simulink model "BLDC_ClosedLoop"  (R2025a)
settings: Solver=FixedStepDiscrete  StartTime=0.0  StopTime=Tsim  FixedStep=Ts  RelTol=1e-3
undefined symbols (not defined in the file): antiWindupEnable, B, DiscIntNeverNeededParam, fPWM, J, Ki, Kp, Ls, polePairs, refSpeed1, refSpeed2, refTime1, refTime2, Rs, speedRampRate, TloadInitial, TloadStep, TloadStepTime, Ts, Ts_speed, uMax, uMin, Vdc
libraries: simulink x7, spsPermanentMagnetSynchronousMachineLib x1, spsControlledVoltageSourceLib x1, spsUniversalBridgeLib x1, spsVoltageMeasurementLib x1, spspowerguiLib x1
settings Model: Creator=yegan  LastModifiedBy=yegan
settings SolverCC: AutoInsertRateTranBlk=on
settings DataIOCC: SaveOutput=off  SaveTime=off

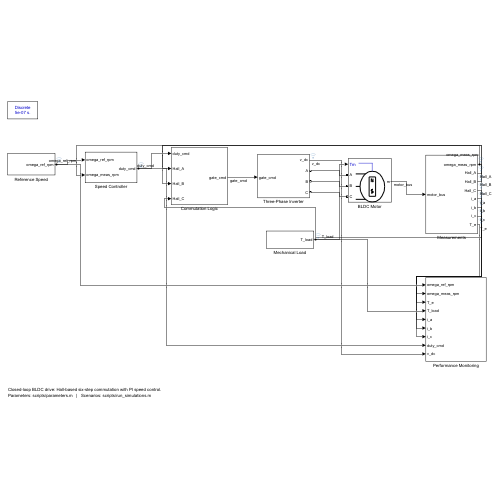
[thumbnail: Simulink's stored preview of the top-level diagram]
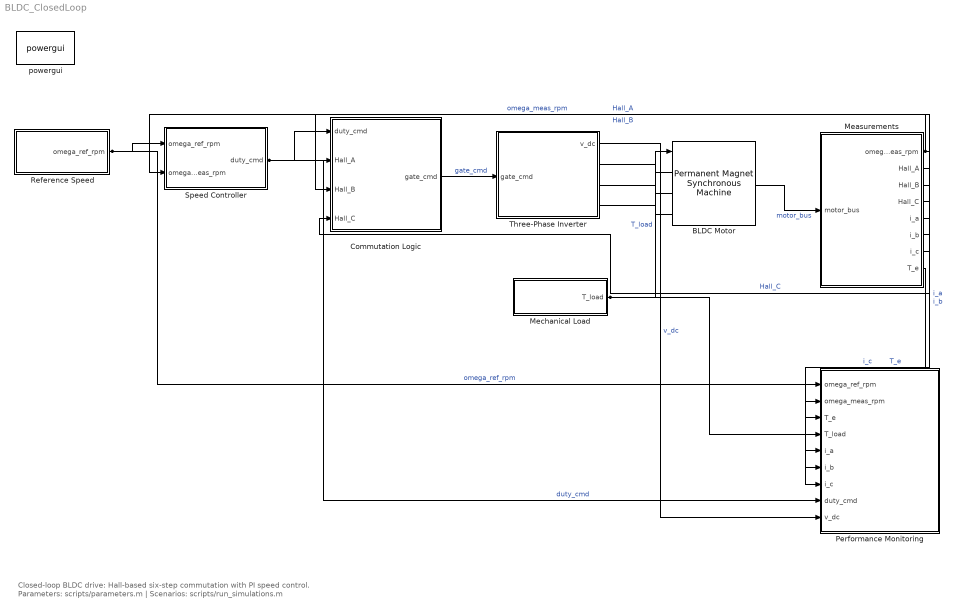
== system BLDC_ClosedLoop ==
  note: Closed-loop BLDC drive: Hall-based six-step commutation with PI speed control.
      | Parameters: scripts/parameters.m   |   Scenarios: scripts/run_simulations.m
  BLDC Motor : spsPermanentMagnetSynchronousMachineLib/Permanent Magnet Synchronous Machine  NbPhases=3  FluxDistribution=Trapezoidal  RotorType=Round  MechanicalLoad=Torque Tm  PresetModel=No  ShowDetailedParameters=on  MeasurementBus=off  Resistance=Rs  Inductance=Ls  dqInductances=[8.5e-3,8.5e-3]  La=0.000395  MachineConstant=Flux linkage established by magnets (V.s)  Flux=fluxPM  VoltageCst=87.9646  TorqueCst=0.84  Flat=flatTopDeg  Mechanical=[J, B, polePairs, 0]  PolePairs=polePairs  InitialConditions=[0, 0, 0, 0]  InitialConditions5ph=[0 0 0 0 0 0]  RefAngle=90 degrees behind phase A axis (modified Park)  IterativeDiscreteModel=Trapezoidal non iterative  TsBlock=-1  TsPowergui=0
  Commutation Logic : Subsystem
  Measurements : Subsystem
  Mechanical Load : Subsystem
  Performance Monitoring : Subsystem
  Reference Speed : Subsystem
  Speed Controller : Subsystem
  Three-Phase Inverter : Subsystem
  powergui : spspowerguiLib/powergui  Priority=1  SimulationMode=Discrete  SampleTime=Ts  frequency=60  Iterations=50  frequencyindice=60  Pbase=100e6  ErrMax=1e-4  UnitsV=kV  UnitsW=MW  buscounter=0  FunctionMessages=off  echomessages=off  EnableUseOfTLC=off  CurrentSourceSwitches=off  DisableSnubberDevices=off  DisableRonSwitches=off  DisableVfSwitches=off  DisplayEquations=off  AutomaticDiscreteSolvers=off  SolverType=Tustin/Backward Euler (TBE)  Interpol=off  ExternalGateDelay=off  methode=off  Ts=100  x0status=blocks  SPID=on  SwTol=0  HookPort=off  NonlinearTolerance=1e-4  nMaxIteration=100  ContinueOnMaxIteration=off  RestoreLinks=warning  ResistiveCurrentMeasurement=off  Frange=[0:2:500]  Ylog=off  Xlog=on  ShowGrid=off  save=off  variable=ZData  structure=0  ZoomFFT=off  StartTime=0.0  cycles=1  DisplayStyle=1  fundamental=60  FreqAxis=off  MaxFrequency=1000  frequencyindicesteady=1  RmsSteady=1  display=off
  wires:
  Reference Speed/1(omega_ref_rpm) -> Speed Controller/1(omega_ref_rpm), Performance Monitoring/1(omega_ref_rpm)  "omega_ref_rpm"
  Speed Controller/1(duty_cmd) -> Commutation Logic/1(duty_cmd), Performance Monitoring/8(duty_cmd)  "duty_cmd"
  Commutation Logic/1(gate_cmd) -> Three-Phase Inverter/1(gate_cmd)  "gate_cmd"
  Three-Phase Inverter/1(v_dc) -> Performance Monitoring/9(v_dc)  "v_dc"
  Mechanical Load/1(T_load) -> BLDC Motor/1, Performance Monitoring/4(T_load)  "T_load"
  BLDC Motor/1 -> Measurements/1(motor_bus)  "motor_bus"
  Measurements/1(omega_meas_rpm) -> Speed Controller/2(omega_meas_rpm), Performance Monitoring/2(omega_meas_rpm)  "omega_meas_rpm"
  Measurements/2(Hall_A) -> Commutation Logic/2(Hall_A)  "Hall_A"
  Measurements/3(Hall_B) -> Commutation Logic/3(Hall_B)  "Hall_B"
  Measurements/4(Hall_C) -> Commutation Logic/4(Hall_C)  "Hall_C"
  Measurements/5(i_a) -> Performance Monitoring/5(i_a)  "i_a"
  Measurements/6(i_b) -> Performance Monitoring/6(i_b)  "i_b"
  Measurements/7(i_c) -> Performance Monitoring/7(i_c)  "i_c"
  Measurements/8(T_e) -> Performance Monitoring/3(T_e)  "T_e"
  connections:
  Three-Phase Inverter/RConn1 -- BLDC Motor/LConn1
  Three-Phase Inverter/RConn2 -- BLDC Motor/LConn2
  Three-Phase Inverter/RConn3 -- BLDC Motor/LConn3

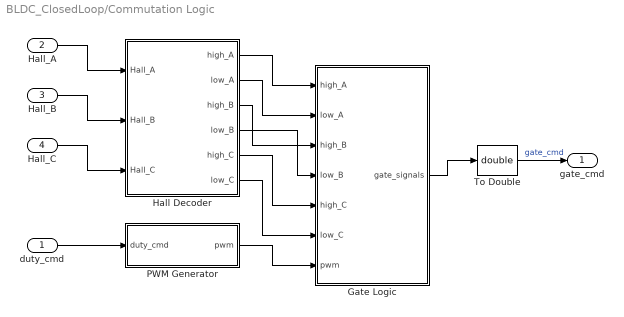
== system BLDC_ClosedLoop/Commutation Logic ==
  duty_cmd : Inport
  Hall_A : Inport  Port=2
  Hall_B : Inport  Port=3
  Hall_C : Inport  Port=4
  Gate Logic : Subsystem
  Hall Decoder : Subsystem
  PWM Generator : Subsystem
  To Double : DataTypeConversion  OutDataTypeStr=double  SaturateOnIntegerOverflow=off  RndMeth=Floor
  gate_cmd : Outport
  wires:
  Hall_A/1 -> Hall Decoder/1(Hall_A)
  Hall_B/1 -> Hall Decoder/2(Hall_B)
  Hall_C/1 -> Hall Decoder/3(Hall_C)
  duty_cmd/1 -> PWM Generator/1(duty_cmd)
  Hall Decoder/1(high_A) -> Gate Logic/1(high_A)
  Hall Decoder/2(low_A) -> Gate Logic/2(low_A)
  Hall Decoder/3(high_B) -> Gate Logic/3(high_B)
  Hall Decoder/4(low_B) -> Gate Logic/4(low_B)
  Hall Decoder/5(high_C) -> Gate Logic/5(high_C)
  Hall Decoder/6(low_C) -> Gate Logic/6(low_C)
  PWM Generator/1(pwm) -> Gate Logic/7(pwm)
  Gate Logic/1(gate_signals) -> To Double/1
  To Double/1 -> gate_cmd/1  "gate_cmd"

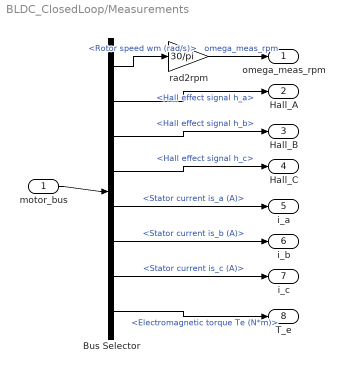
== system BLDC_ClosedLoop/Measurements ==
  motor_bus : Inport
  Bus Selector : BusSelector  OutputSignals=Rotor speed wm (rad/s),Hall effect signal h_a,Hall effect signal h_b,Hall effect signal h_c,Stator current is_a (A),Stator current is_b (A),Stator current is_c (A),Electromagnetic torque Te (N*m)
  rad2rpm : Gain  Gain=30/pi
  omega_meas_rpm : Outport
  Hall_A : Outport  Port=2
  Hall_B : Outport  Port=3
  Hall_C : Outport  Port=4
  i_a : Outport  Port=5
  i_b : Outport  Port=6
  i_c : Outport  Port=7
  T_e : Outport  Port=8
  wires:
  motor_bus/1 -> Bus Selector/1
  Bus Selector/1 -> rad2rpm/1  "<Rotor speed wm (rad/s)>"
  rad2rpm/1 -> omega_meas_rpm/1  "omega_meas_rpm"
  Bus Selector/2 -> Hall_A/1  "<Hall effect signal h_a>"
  Bus Selector/3 -> Hall_B/1  "<Hall effect signal h_b>"
  Bus Selector/4 -> Hall_C/1  "<Hall effect signal h_c>"
  Bus Selector/5 -> i_a/1  "<Stator current is_a (A)>"
  Bus Selector/6 -> i_b/1  "<Stator current is_b (A)>"
  Bus Selector/7 -> i_c/1  "<Stator current is_c (A)>"
  Bus Selector/8 -> T_e/1  "<Electromagnetic torque Te (N*m)>"

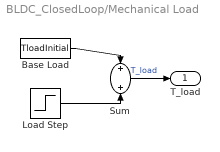
== system BLDC_ClosedLoop/Mechanical Load ==
  Base Load : Constant  Value=TloadInitial
  Load Step : Step  Time=TloadStepTime  After=TloadStep  SampleTime=0
  Sum : Sum
  T_load : Outport
  wires:
  Base Load/1 -> Sum/1
  Load Step/1 -> Sum/2
  Sum/1 -> T_load/1  "T_load"

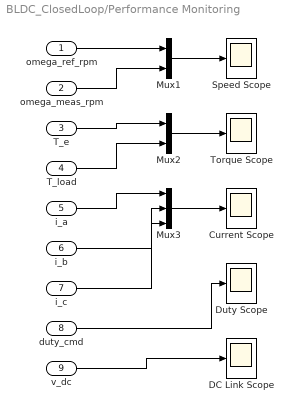
== system BLDC_ClosedLoop/Performance Monitoring ==
  omega_ref_rpm : Inport
  omega_meas_rpm : Inport  Port=2
  T_e : Inport  Port=3
  T_load : Inport  Port=4
  i_a : Inport  Port=5
  i_b : Inport  Port=6
  i_c : Inport  Port=7
  duty_cmd : Inport  Port=8
  v_dc : Inport  Port=9
  Current Scope : Scope
  DC Link Scope : Scope
  Duty Scope : Scope
  Mux1 : Mux  Inputs=2
  Mux2 : Mux  Inputs=2
  Mux3 : Mux  Inputs=3
  Speed Scope : Scope
  Torque Scope : Scope
  wires:
  omega_ref_rpm/1 -> Mux1/1
  omega_meas_rpm/1 -> Mux1/2
  Mux1/1 -> Speed Scope/1
  T_e/1 -> Mux2/1
  T_load/1 -> Mux2/2
  Mux2/1 -> Torque Scope/1
  i_a/1 -> Mux3/1
  i_b/1 -> Mux3/2
  i_c/1 -> Mux3/3
  Mux3/1 -> Current Scope/1
  duty_cmd/1 -> Duty Scope/1
  v_dc/1 -> DC Link Scope/1

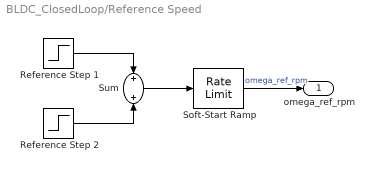
== system BLDC_ClosedLoop/Reference Speed ==
  Reference Step 1 : Step  Time=refTime1  After=refSpeed1  SampleTime=Ts_speed
  Reference Step 2 : Step  Time=refTime2  After=refSpeed2 - refSpeed1  SampleTime=Ts_speed
  Soft-Start Ramp : RateLimiter  RisingSlewLimit=speedRampRate  FallingSlewLimit=-speedRampRate  SampleTimeMode=inherited
  Sum : Sum
  omega_ref_rpm : Outport
  wires:
  Reference Step 1/1 -> Sum/1
  Reference Step 2/1 -> Sum/2
  Sum/1 -> Soft-Start Ramp/1
  Soft-Start Ramp/1 -> omega_ref_rpm/1  "omega_ref_rpm"

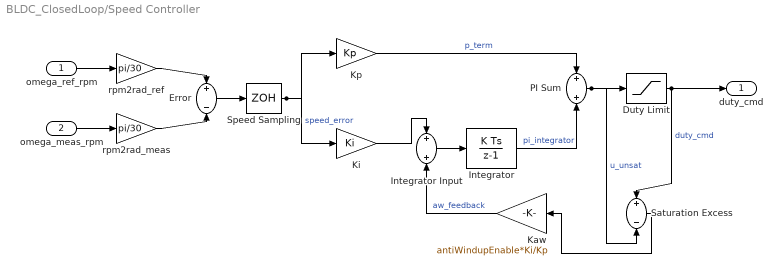
== system BLDC_ClosedLoop/Speed Controller ==
  omega_ref_rpm : Inport
  omega_meas_rpm : Inport  Port=2
  Duty Limit : Saturate  UpperLimit=uMax  LowerLimit=uMin
  Error : Sum  Inputs=+-
  Integrator : DiscreteIntegrator  SampleTime=-1  ICPrevOutput=DiscIntNeverNeededParam  ICPrevScaledInput=DiscIntNeverNeededParam
  Integrator Input : Sum
  Kaw : Gain  Gain=antiWindupEnable*Ki/Kp
  Ki : Gain  Gain=Ki
  Kp : Gain  Gain=Kp
  PI Sum : Sum
  Saturation Excess : Sum  Inputs=+-
  Speed Sampling : ZeroOrderHold  SampleTime=Ts_speed
  rpm2rad_meas : Gain  Gain=pi/30
  rpm2rad_ref : Gain  Gain=pi/30
  duty_cmd : Outport
  wires:
  omega_ref_rpm/1 -> rpm2rad_ref/1
  omega_meas_rpm/1 -> rpm2rad_meas/1
  rpm2rad_ref/1 -> Error/1
  rpm2rad_meas/1 -> Error/2
  Error/1 -> Speed Sampling/1
  Speed Sampling/1 -> Kp/1, Ki/1  "speed_error"
  Ki/1 -> Integrator Input/1
  Integrator Input/1 -> Integrator/1
  Integrator/1 -> PI Sum/2  "pi_integrator"
  Kp/1 -> PI Sum/1  "p_term"
  PI Sum/1 -> Duty Limit/1, Saturation Excess/2  "u_unsat"
  Duty Limit/1 -> duty_cmd/1, Saturation Excess/1  "duty_cmd"
  Saturation Excess/1 -> Kaw/1
  Kaw/1 -> Integrator Input/2  "aw_feedback"

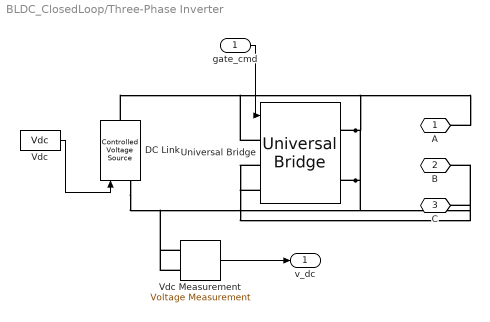
== system BLDC_ClosedLoop/Three-Phase Inverter ==
  gate_cmd : Inport
  DC Link : spsControlledVoltageSourceLib/Controlled Voltage Source  Initialize=on  Source_Type=DC  Amplitude=Vdc  Phase=0  Frequency=0  Measurements=None
  Universal Bridge : spsUniversalBridgeLib/Universal Bridge  Arms=3  SnubberResistance=Rsnubber  SnubberCapacitance=Csnubber  Device=MOSFET / Diodes  Ron=Ron  Lon=0  ForwardVoltages="[  0  0  ]"  ForwardVoltage=0  GTOparameters=[ 10e-6 , 20e-6 ]  IGBTparameters=[ 1e-6 , 2e-6 ]  Measurements=None  Measurements_2=None  converterType=Rectifier
  Vdc : Constant  Value=Vdc
  Vdc Measurement : spsVoltageMeasurementLib/Voltage Measurement  PhasorSimulation=off  OutputType=Complex  PSBequivalent=0
  A : PMIOPort  Side=Right
  B : PMIOPort  Port=2  Side=Right
  C : PMIOPort  Port=3  Side=Right
  v_dc : Outport
  wires:
  Vdc/1 -> DC Link/1
  gate_cmd/1 -> Universal Bridge/1
  Vdc Measurement/1 -> v_dc/1
  connections:
  Universal Bridge/RConn1 -- DC Link/RConn1 -- Vdc Measurement/LConn1
  Universal Bridge/RConn2 -- DC Link/LConn1 -- Vdc Measurement/LConn2
  Universal Bridge/LConn1 -- A/RConn1
  Universal Bridge/LConn2 -- B/RConn1
  Universal Bridge/LConn3 -- C/RConn1

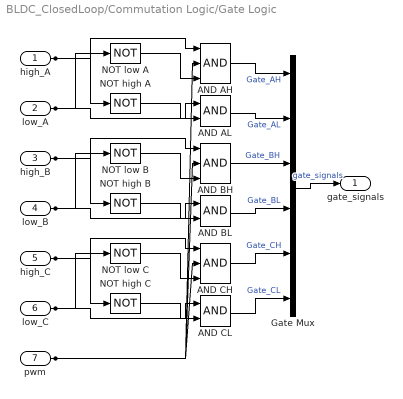
== system BLDC_ClosedLoop/Commutation Logic/Gate Logic ==
  high_A : Inport
  low_A : Inport  Port=2
  high_B : Inport  Port=3
  low_B : Inport  Port=4
  high_C : Inport  Port=5
  low_C : Inport  Port=6
  pwm : Inport  Port=7
  AND AH : Logic  Inputs=3  AllPortsSameDT=off  OutDataTypeStr=boolean
  AND AL : Logic  AllPortsSameDT=off  OutDataTypeStr=boolean
  AND BH : Logic  Inputs=3  AllPortsSameDT=off  OutDataTypeStr=boolean
  AND BL : Logic  AllPortsSameDT=off  OutDataTypeStr=boolean
  AND CH : Logic  Inputs=3  AllPortsSameDT=off  OutDataTypeStr=boolean
  AND CL : Logic  AllPortsSameDT=off  OutDataTypeStr=boolean
  Gate Mux : Mux  Inputs=6
  NOT high A : Logic  Operator=NOT  AllPortsSameDT=off  OutDataTypeStr=boolean
  NOT high B : Logic  Operator=NOT  AllPortsSameDT=off  OutDataTypeStr=boolean
  NOT high C : Logic  Operator=NOT  AllPortsSameDT=off  OutDataTypeStr=boolean
  NOT low A : Logic  Operator=NOT  AllPortsSameDT=off  OutDataTypeStr=boolean
  NOT low B : Logic  Operator=NOT  AllPortsSameDT=off  OutDataTypeStr=boolean
  NOT low C : Logic  Operator=NOT  AllPortsSameDT=off  OutDataTypeStr=boolean
  gate_signals : Outport
  wires:
  low_A/1 -> NOT low A/1, AND AL/1
  high_A/1 -> NOT high A/1, AND AH/1
  pwm/1 -> AND AH/2, AND BH/2, AND CH/2
  NOT low A/1 -> AND AH/3
  NOT high A/1 -> AND AL/2
  low_B/1 -> NOT low B/1, AND BL/1
  high_B/1 -> NOT high B/1, AND BH/1
  NOT low B/1 -> AND BH/3
  NOT high B/1 -> AND BL/2
  low_C/1 -> NOT low C/1, AND CL/1
  high_C/1 -> NOT high C/1, AND CH/1
  NOT low C/1 -> AND CH/3
  NOT high C/1 -> AND CL/2
  AND AH/1 -> Gate Mux/1  "Gate_AH"
  AND AL/1 -> Gate Mux/2  "Gate_AL"
  AND BH/1 -> Gate Mux/3  "Gate_BH"
  AND BL/1 -> Gate Mux/4  "Gate_BL"
  AND CH/1 -> Gate Mux/5  "Gate_CH"
  AND CL/1 -> Gate Mux/6  "Gate_CL"
  Gate Mux/1 -> gate_signals/1  "gate_signals"

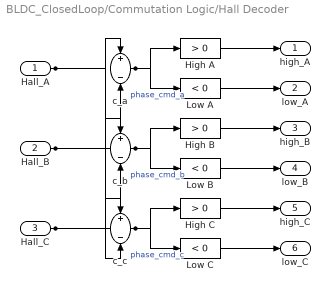
== system BLDC_ClosedLoop/Commutation Logic/Hall Decoder ==
  Hall_A : Inport
  Hall_B : Inport  Port=2
  Hall_C : Inport  Port=3
  High A : simulink/Logic and Bit Operations/Compare To Zero  relop=>  OutDataTypeStr=boolean
  High B : simulink/Logic and Bit Operations/Compare To Zero  relop=>  OutDataTypeStr=boolean
  High C : simulink/Logic and Bit Operations/Compare To Zero  relop=>  OutDataTypeStr=boolean
  Low A : simulink/Logic and Bit Operations/Compare To Zero  relop=<  OutDataTypeStr=boolean
  Low B : simulink/Logic and Bit Operations/Compare To Zero  relop=<  OutDataTypeStr=boolean
  Low C : simulink/Logic and Bit Operations/Compare To Zero  relop=<  OutDataTypeStr=boolean
  c_a : Sum  Inputs=+-
  c_b : Sum  Inputs=+-
  c_c : Sum  Inputs=+-
  high_A : Outport
  low_A : Outport  Port=2
  high_B : Outport  Port=3
  low_B : Outport  Port=4
  high_C : Outport  Port=5
  low_C : Outport  Port=6
  wires:
  Hall_A/1 -> c_a/1, c_c/2
  Hall_B/1 -> c_a/2, c_b/1
  c_a/1 -> High A/1, Low A/1  "phase_cmd_a"
  High A/1 -> high_A/1
  Low A/1 -> low_A/1
  Hall_C/1 -> c_b/2, c_c/1
  c_b/1 -> High B/1, Low B/1  "phase_cmd_b"
  High B/1 -> high_B/1
  Low B/1 -> low_B/1
  c_c/1 -> High C/1, Low C/1  "phase_cmd_c"
  High C/1 -> high_C/1
  Low C/1 -> low_C/1

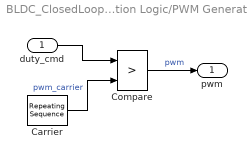
== system BLDC_ClosedLoop/Commutation Logic/PWM Generator ==
  duty_cmd : Inport
  Carrier : simulink/Sources/Repeating Sequence  rep_seq_t=[0 0.5 1]/fPWM  rep_seq_y=[0 1 0]
  Compare : RelationalOperator  Operator=>  OutDataTypeStr=boolean  RndMeth=Simplest  InputSameDT=off
  pwm : Outport
  wires:
  duty_cmd/1 -> Compare/1
  Carrier/1 -> Compare/2  "pwm_carrier"
  Compare/1 -> pwm/1  "pwm"
